simulink model "ACEServoCard"  (R2025b)
settings: Solver=ode4  StartTime=0.0  StopTime=inf  FixedStep=0.01  RelTol=1e-3
undefined symbols (not defined in the file or in its folder): RS422, TTL, UART4, UART5
libraries: AFCToolbox x9, simulink x1
settings Model: Creator=zqinghua  LastModifiedBy=zqhkd
settings OptimizationCC: DefaultParameterBehavior=Inlined  EnhancedBackFolding=on  PassReuseOutputArgsAs=Individual arguments  ZeroExternalMemoryAtStartup=off  ZeroInternalMemoryAtStartup=off  OptimizeBlockOrder=speed  DifferentSizesBufferReuse=on  OptimizationCustomize=off  EfficientTunableParamExpr=on
settings DebuggingCC: ParameterTunabilityLossMsg=error
settings HardwareCC: ProdBitPerInt=16.0  ProdBitPerPointer=16.0  ProdBitPerSizeT=16.0  ProdBitPerPtrDiffT=16.0  ProdLargestAtomicFloat=None  ProdWordSize=16.0  ProdHWDeviceType=STMicroelectronics->ST10/Super10
settings SFSimCC: MATLABDynamicMemAlloc=off
settings RTWCC: SystemTargetFile=AFCHawk.tlc  GenCodeOnly=on  TemplateMakefile=ert_default_tmf  GPUComputeCapability=3.5  Description=Embedded Coder
settings CodeAppCC: ForceParamTrailComments=on  IgnoreCustomStorageClasses=off  OperatorAnnotations=on  SimulinkDataObjDesc=on  SFDataObjDesc=on  InsertBlockDesc=on
settings STFCustomTargetCC: SystemTargetFile=AFCHawk.tlc  TargetLangStandard=C99 (ISO)  MultiwordLength=256.0  ModelReferenceCompliant=off  ConcurrentExecutionCompliant=off  CombineOutputUpdateFcns=on  ERTCustomFileBanners=on  SupportContinuousTime=off  SupportNonInlinedSFcns=off  RemoveResetFunc=on  MATLABClassNameForMDSCustomization=Simulink.SoftwareTarget.ERTCustomization  GRTInterface=off  t_DownLoad2Target=on  t_comPort=2.0  t_BuildCPrj2Hex=on  t_comBaud=460800.0
settings ERTTargetCC: ERTCustomFileTemplate=example_file_process.tlc  DynamicArrayContainerType=coder::array  TargetLangStandard=C99 (ISO)  ModelReferenceCompliant=off  ParMdlRefBuildCompliant=off  CompOptLevelCompliant=off  ConcurrentExecutionCompliant=off  ModelStepFunctionPrototypeControlCompliant=off  CPPClassGenCompliant=off  UseToolchainInfoCompliant=off

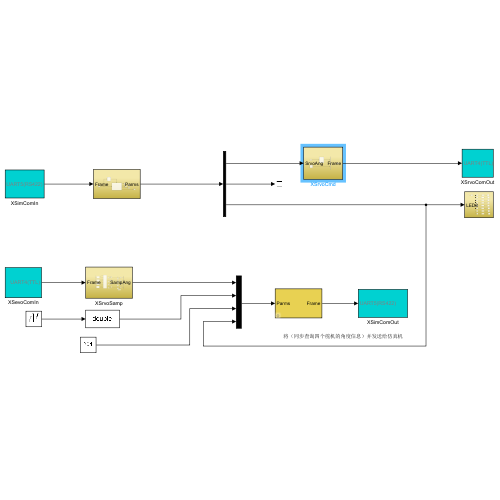
[thumbnail: Simulink's stored preview of the top-level diagram]
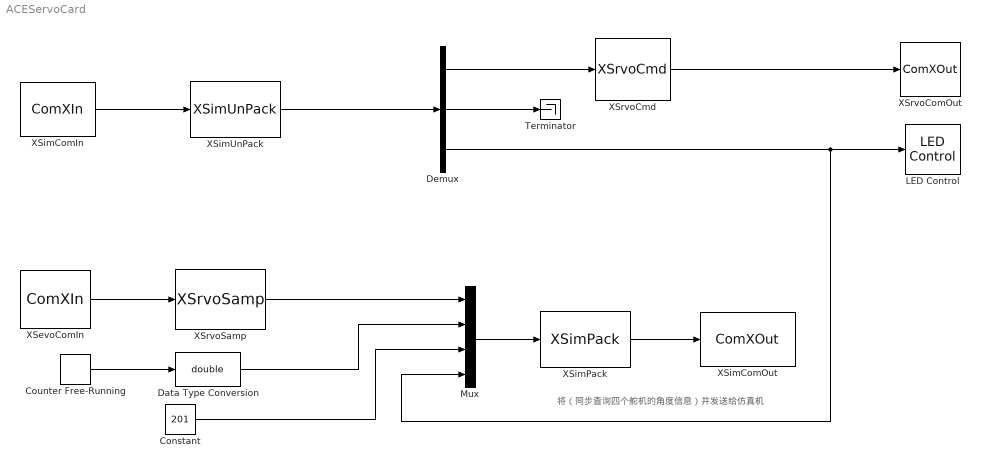
== system ACEServoCard ==
  note: 将（同步查询四个舵机的角度信息）并发送给仿真机
  Constant : Constant  Value=201
  Counter Free-Running : simulink/Sources/Counter Free-Running  NumBits=32  tsamp=-1
  Data Type Conversion : DataTypeConversion  OutDataTypeStr=double  SaturateOnIntegerOverflow=off  RndMeth=Floor
  Demux : Demux  Outputs=[4,2,1]
  LED Control : AFCToolbox/ServoCardModule/LED Control  SystemSampleTime=-1  VariantActivationTime=update diagram  EmptyChoice=off  PassThrough=off  PassThroughVariantControl=(default)  EmptyChoiceVariantControl=(default)  AllowFlexibleInterface=on  Latency=0  AutoFrameSizeCalculation=off
      settings: SourceProductName=AFCToolbox
  Mux : Mux
  Terminator : Terminator
  XSevoComIn : AFCToolbox/DeviceModule/ComXIn  Priority=2  g_sampleTime=0.01  g_comPort=UART4(TTL)  g_baudRate=1000000  g_dataSize=4*8  g_parity=0  g_stopBits=1
      settings: SourceProductName=AFCToolbox
  XSimComIn : AFCToolbox/DeviceModule/ComXIn  Priority=2  g_sampleTime=0.01  g_comPort=UART5(RS422)  g_baudRate=460800  g_dataSize=40  g_parity=0  g_stopBits=1
      settings: SourceProductName=AFCToolbox
  XSimComOut : AFCToolbox/DeviceModule/ComXOut  Priority=8  g_comPort=UART5(RS422)  g_baudRate=460800  g_outFreq=1
      settings: SourceProductName=AFCToolbox
  XSimPack : AFCToolbox/ServoCardModule/XSimPack  frameSender=0  frameType=80
      settings: SourceProductName=AFCToolbox
  XSimUnPack : AFCToolbox/ServoCardModule/XSimUnPack  SystemSampleTime=-1  VariantActivationTime=update diagram  EmptyChoice=off  PassThrough=off  PassThroughVariantControl=(default)  EmptyChoiceVariantControl=(default)  AllowFlexibleInterface=on  Latency=0  AutoFrameSizeCalculation=off
      settings: SourceProductName=AFCToolbox
  XSrvoCmd : AFCToolbox/ServoCardModule/XSrvoCmd  SystemSampleTime=-1  VariantActivationTime=update diagram  EmptyChoice=off  PassThrough=off  PassThroughVariantControl=(default)  EmptyChoiceVariantControl=(default)  AllowFlexibleInterface=on  Latency=0  AutoFrameSizeCalculation=off
      settings: SourceProductName=AFCToolbox
  XSrvoComOut : AFCToolbox/DeviceModule/ComXOut  Priority=8  g_comPort=UART4(TTL)  g_baudRate=1000000  g_outFreq=1
      settings: SourceProductName=AFCToolbox
  XSrvoSamp : AFCToolbox/ServoCardModule/XSrvoSamp  SystemSampleTime=-1  VariantActivationTime=update diagram  EmptyChoice=off  PassThrough=off  PassThroughVariantControl=(default)  EmptyChoiceVariantControl=(default)  AllowFlexibleInterface=on  Latency=0  AutoFrameSizeCalculation=off
      settings: SourceProductName=AFCToolbox
  wires:
  Demux/2 -> Terminator/1
  Demux/1 -> XSrvoCmd/1
  Demux/3 -> LED Control/1, Mux/4
  XSevoComIn/1 -> XSrvoSamp/1
  XSrvoSamp/1 -> Mux/1
  Mux/1 -> XSimPack/1
  XSimPack/1 -> XSimComOut/1
  XSrvoCmd/1 -> XSrvoComOut/1
  Counter Free-Running/1 -> Data Type Conversion/1
  Data Type Conversion/1 -> Mux/2
  Constant/1 -> Mux/3
  XSimComIn/1 -> XSimUnPack/1
  XSimUnPack/1 -> Demux/1
